simulink model "Artificial_Pancreas_Control"  (R2017a)
settings: Solver=VariableStepAuto  StartTime=0.0  StopTime=200  RelTol=1e-3
libraries: simulink x1
settings Model: Creator=USER  LastModifiedBy=USER

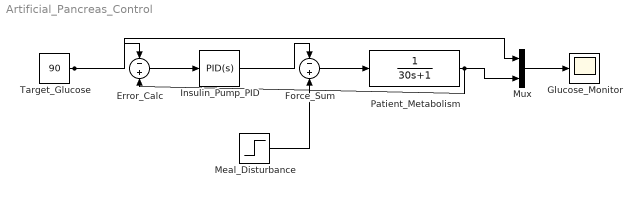
== system Artificial_Pancreas_Control ==
  Error_Calc : Sum  Inputs=-|+
  Force_Sum : Sum  Inputs=-|+
  Glucose_Monitor : Scope
  Insulin_Pump_PID : simulink/Continuous/PID Controller  Controller=PID  TimeDomain=Continuous-time  SampleTime=-1  IntegratorMethod=Forward Euler  FilterMethod=Forward Euler  Form=Parallel  UseFilter=on  ControllerParametersSource=internal  P=1.5  I=0.05  D=2.0  N=100  InitialConditionSource=internal  InitialConditionForIntegrator=0  InitialConditionForFilter=0  ExternalReset=none  LimitOutput=off  UpperSaturationLimit=inf  LowerSaturationLimit=-inf  LinearizeAsGain=on  AntiWindupMode=none  Kb=1  TrackingMode=off  Kt=1  PParamMin=[]  PParamMax=[]  IParamMin=[]  IParamMax=[]  DParamMin=[]  DParamMax=[]  NParamMin=[]  NParamMax=[]  KbParamMin=[]  KbParamMax=[]  KtParamMin=[]  KtParamMax=[]  POutMin=[]  POutMax=[]  IOutMin=[]  IOutMax=[]  DOutMin=[]  DOutMax=[]  NOutMin=[]  NOutMax=[]  KbOutMin=[]  KbOutMax=[]  KtOutMin=[]  KtOutMax=[]  IntegratorOutMin=[]  IntegratorOutMax=[]  FilterOutMin=[]  FilterOutMax=[]  SumOutMin=[]  SumOutMax=[]  SumI1OutMin=[]  SumI1OutMax=[]  SumI2OutMin=[]  SumI2OutMax=[]  SumI3OutMin=[]  SumI3OutMax=[]  SumDOutMin=[]  SumDOutMax=[]  SaturationOutMin=[]  SaturationOutMax=[]  IntegratorContinuousStateAttributes=''  IntegratorStateMustResolveToSignalObject=off  IntegratorRTWStateStorageClass=Auto  FilterContinuousStateAttributes=''  FilterStateMustResolveToSignalObject=off  FilterRTWStateStorageClass=Auto  DifferentiatorICPrevScaledInput=0  DifferentiatorOutMin=[]  DifferentiatorOutMax=[]  InitialConditionSetting=State (most efficient)
  Meal_Disturbance : Step  Time=60  Before=90  After=140  SampleTime=0
  Mux : Mux  Inputs=2
  Patient_Metabolism : TransferFcn  Denominator=[30 1]
  Target_Glucose : Constant  Value=90
  wires:
  Target_Glucose/1 -> Error_Calc/1, Mux/1
  Patient_Metabolism/1 -> Error_Calc/2, Mux/2
  Error_Calc/1 -> Insulin_Pump_PID/1
  Insulin_Pump_PID/1 -> Force_Sum/1
  Meal_Disturbance/1 -> Force_Sum/2
  Force_Sum/1 -> Patient_Metabolism/1
  Mux/1 -> Glucose_Monitor/1
